simulink model "oscillating_circuit_simulation"  (R2026a)
settings: Solver=ode1  FixedStep=0.001
values from neighbouring files (symbols this model uses):
  C = 16 * 10 ^ -6    (= 1.6e-05)    [parameters.m]
  i_o = 0.1    [parameters.m]
  L = 160    [parameters.m]
  R = 100    [parameters.m]
  U_o = 15    [parameters.m]
settings Model: Creator=coolm  LastModifiedBy=coolm

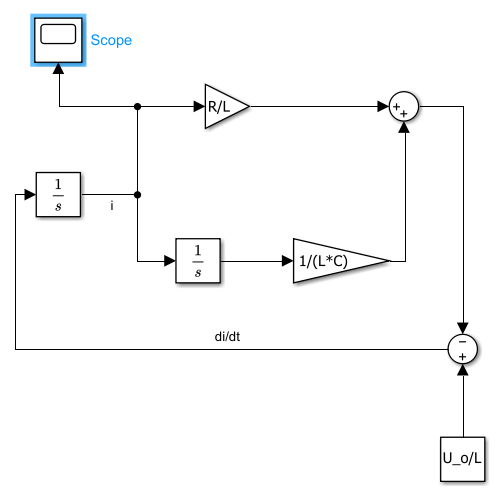
[thumbnail: Simulink's stored preview of the top-level diagram]
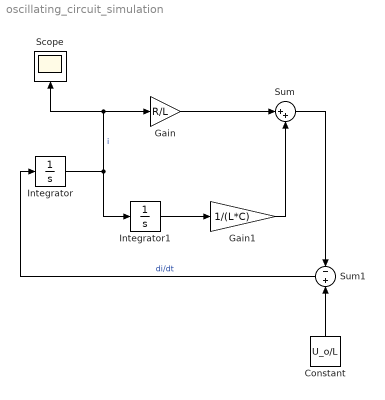
== system oscillating_circuit_simulation ==
  Constant : Constant  Value=U_o/L
  Gain : Gain  Gain=R/L
  Gain1 : Gain  Gain=1/(L*C)
  Integrator : Integrator  InitialCondition=i_o
  Integrator1 : Integrator
  Scope : Scope
      settings: ActiveDisplayYMinimum=-0.35175078825313016  ActiveDisplayYMaximum=0.3901721653015639
  Sum : Sum  Inputs=|++
  Sum1 : Sum  Inputs=-+
  wires:
  Integrator/1 -> Integrator1/1, Scope/1, Gain/1  "i"
  Integrator1/1 -> Gain1/1
  Gain1/1 -> Sum/2
  Gain/1 -> Sum/1
  Sum/1 -> Sum1/1
  Sum1/1 -> Integrator/1  "di/dt"
  Constant/1 -> Sum1/2
